simulink library "sm_car_testrig_utilities_lib"  (R2025a)
settings: Solver=VariableStepAuto  StartTime=0.0  StopTime=10.0  RelTol=1e-3
undefined symbols (not defined in the file): Maneuver, tire_radius, Vehicle, Visual, X, Y, Z
libraries: sm_lib x31, nesl_utility x18, fl_lib x3, $bdroot x3, Tire_Utilities x2, Surface_Profile_Axle2_KnC x2, simulink x2
(part 2 of 2)

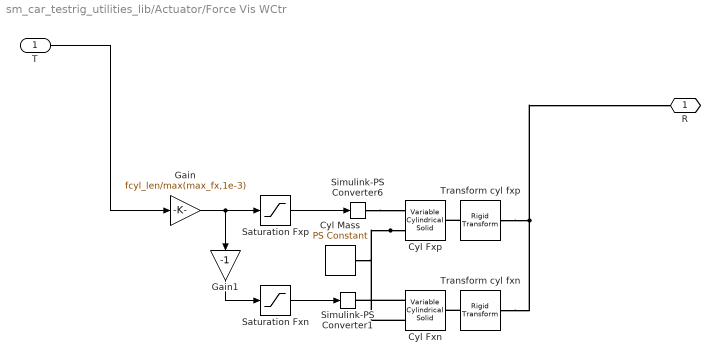
== system sm_car_testrig_utilities_lib/Actuator/Force Vis WCtr ==
  T : Inport
  Cyl Fxn : sm_lib/Body Elements/Variable Mass/Variable Cylindrical Solid  RadiusType=Constant  Radius=fcyl_rad  RadiusUnits=m  LengthType=ProvidedByInput  Length=1e-3  LengthUnits=m  MassType=ProvidedByInput  Density=1000  DensityUnits=kg/m^3  SenseRadius=off  SenseLength=off  SenseMass=off  SenseCenterOfMass=off  SenseInertiaMatrix=off  GraphicType=FromGeometry  MarkerShape=Sphere  MarkerSize=10  GraphicVisPropType=SimpleVisualProperties  GraphicDiffuseColor=fcyl_clr  GraphicOpacity=fcyl_opc  GraphicSpecularColor=[0.5 0.5 0.5 1.0]  GraphicAmbientColor=[0.15 0.15 0.15 1.0]  GraphicEmissiveColor=[0.0 0.0 0.0 1.0]  GraphicShininess=75
  Cyl Fxp : sm_lib/Body Elements/Variable Mass/Variable Cylindrical Solid  RadiusType=Constant  Radius=fcyl_rad  RadiusUnits=m  LengthType=ProvidedByInput  Length=1e-3  LengthUnits=m  MassType=ProvidedByInput  Density=1000  DensityUnits=kg/m^3  SenseRadius=off  SenseLength=off  SenseMass=off  SenseCenterOfMass=off  SenseInertiaMatrix=off  GraphicType=FromGeometry  MarkerShape=Sphere  MarkerSize=10  GraphicVisPropType=SimpleVisualProperties  GraphicDiffuseColor=fcyl_clr  GraphicOpacity=fcyl_opc  GraphicSpecularColor=[0.5 0.5 0.5 1.0]  GraphicAmbientColor=[0.15 0.15 0.15 1.0]  GraphicEmissiveColor=[0.0 0.0 0.0 1.0]  GraphicShininess=75
  Cyl Mass : fl_lib/Physical Signals/Sources/PS Constant  constant=1e-3
  Gain : Gain  Gain=fcyl_len/max(max_fx,1e-3)
  Gain1 : Gain  Gain=-1
  Saturation Fxn : Saturate  UpperLimit=inf  LowerLimit=0  ZeroCross=off
  Saturation Fxp : Saturate  UpperLimit=inf  LowerLimit=0  ZeroCross=off
  Simulink-PS Converter1 : nesl_utility/Simulink-PS Converter  PhysicalDomain=network_engine_domain  SubClassName=ps_input  LeftPortType=input  RightPortType=output  PseudoPeriodic=off  Frequencies=[]  NoiseDistribution=none  NoiseParameters=[]  Unit=1  AffineConversion=off  FilteringAndDerivatives=provide  SimscapeFilterOrder=1  InputFilterTimeConstant=0.001  UdotUserProvided=0
  Simulink-PS Converter6 : nesl_utility/Simulink-PS Converter  PhysicalDomain=network_engine_domain  SubClassName=ps_input  LeftPortType=input  RightPortType=output  PseudoPeriodic=off  Frequencies=[]  NoiseDistribution=none  NoiseParameters=[]  Unit=1  AffineConversion=off  FilteringAndDerivatives=provide  SimscapeFilterOrder=1  InputFilterTimeConstant=0.001  UdotUserProvided=0
  Transform cyl fxn : sm_lib/Frames and Transforms/Rigid Transform  RotationMethod=StandardAxis  FollAlignAxisA=+X  BaseAlignAxisA=+Y  FollAlignAxisB=+Y  BaseAlignAxisB=+Z  RotationStandardAxis=+Y  RotationAngle=-90  RotationAngleUnits=deg  RotationArbitraryAxis=[0 0 1]  RotationSequenceAxes=FollowerAxes  RotationSequence=XYX  RotationSequenceAngles=[0 0 0]  RotationSequenceAnglesUnits=deg  RotationMatrix=[1 0 0; 0 1 0; 0 0 1]  Quaternion=[1 0 0 0]  TranslationMethod=None  TranslationCartesianOffset=[0 0 0]  TranslationCartesianOffsetUnits=m  TranslationStandardAxis=+Z  TranslationStandardOffset=0  TranslationStandardOffsetUnits=m  TranslationROffset=0  TranslationROffsetUnits=m  TranslationThetaOffset=0  TranslationThetaOffsetUnits=deg  TranslationZOffset=0  TranslationZOffsetUnits=m
  Transform cyl fxp : sm_lib/Frames and Transforms/Rigid Transform  RotationMethod=StandardAxis  FollAlignAxisA=+X  BaseAlignAxisA=+Y  FollAlignAxisB=+Y  BaseAlignAxisB=+Z  RotationStandardAxis=+Y  RotationAngle=90  RotationAngleUnits=deg  RotationArbitraryAxis=[0 0 1]  RotationSequenceAxes=FollowerAxes  RotationSequence=XYX  RotationSequenceAngles=[0 0 0]  RotationSequenceAnglesUnits=deg  RotationMatrix=[1 0 0; 0 1 0; 0 0 1]  Quaternion=[1 0 0 0]  TranslationMethod=None  TranslationCartesianOffset=[0 0 0]  TranslationCartesianOffsetUnits=m  TranslationStandardAxis=+Z  TranslationStandardOffset=0  TranslationStandardOffsetUnits=m  TranslationROffset=0  TranslationROffsetUnits=m  TranslationThetaOffset=0  TranslationThetaOffsetUnits=deg  TranslationZOffset=0  TranslationZOffsetUnits=m
  R : PMIOPort  Side=Right
  wires:
  Saturation Fxn/1 -> Simulink-PS Converter1/1
  Saturation Fxp/1 -> Simulink-PS Converter6/1
  Gain/1 -> Saturation Fxp/1, Gain1/1
  T/1 -> Gain/1
  Gain1/1 -> Saturation Fxn/1
  connections:
  Cyl Fxp/LConn2 -- Cyl Fxn/LConn2 -- Cyl Mass/RConn1
  Transform cyl fxp/LConn1 -- Transform cyl fxn/LConn1 -- R/RConn1
  Simulink-PS Converter6/RConn1 -- Cyl Fxp/LConn1
  Transform cyl fxp/RConn1 -- Cyl Fxp/RConn1
  Cyl Fxn/LConn1 -- Simulink-PS Converter1/RConn1
  Transform cyl fxn/RConn1 -- Cyl Fxn/RConn1

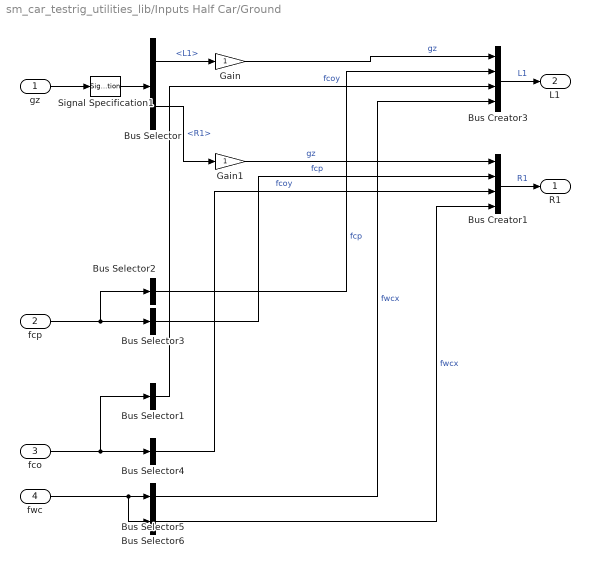
== system sm_car_testrig_utilities_lib/Inputs Half Car/Ground ==
  gz : Inport
  fcp : Inport  Port=2
  fco : Inport  Port=3
  fwc : Inport  Port=4
  Bus Creator1 : BusCreator  Inputs=4
  Bus Creator3 : BusCreator  Inputs=4
  Bus Selector : BusSelector  OutputSignals=L1,R1
  Bus Selector1 : BusSelector  OutputSignals=L1.fcoy  OutputAsBus=on
  Bus Selector2 : BusSelector  OutputSignals=L1.fx,L1.fy,L1.tz  OutputAsBus=on
  Bus Selector3 : BusSelector  OutputSignals=R1.fx,R1.fy,R1.tz  OutputAsBus=on
  Bus Selector4 : BusSelector  OutputSignals=R1.fcoy  OutputAsBus=on
  Bus Selector5 : BusSelector  OutputSignals=L1.fwcx  OutputAsBus=on
  Bus Selector6 : BusSelector  OutputSignals=R1.fwcx  OutputAsBus=on
  Gain : Gain
  Gain1 : Gain
  Signal Specification1 : SignalSpecification  Unit=m
  R1 : Outport  VectorParamsAs1DForOutWhenUnconnected=off
  L1 : Outport  Port=2  VectorParamsAs1DForOutWhenUnconnected=off
  wires:
  Bus Creator1/1 -> R1/1  "R1"
  Bus Creator3/1 -> L1/1  "L1"
  Signal Specification1/1 -> Bus Selector/1
  Bus Selector/1 -> Gain/1  "<L1>"
  gz/1 -> Signal Specification1/1
  Bus Selector/2 -> Gain1/1  "<R1>"
  Gain1/1 -> Bus Creator1/1  "gz"
  Gain/1 -> Bus Creator3/1  "gz"
  Bus Selector3/1 -> Bus Creator1/2  "fcp"
  fcp/1 -> Bus Selector2/1, Bus Selector3/1
  Bus Selector2/1 -> Bus Creator3/2  "fcp"
  fco/1 -> Bus Selector4/1, Bus Selector1/1
  Bus Selector1/1 -> Bus Creator3/3  "fcoy"
  Bus Selector4/1 -> Bus Creator1/3  "fcoy"
  fwc/1 -> Bus Selector6/1, Bus Selector5/1
  Bus Selector5/1 -> Bus Creator3/4  "fwcx"
  Bus Selector6/1 -> Bus Creator1/4  "fwcx"

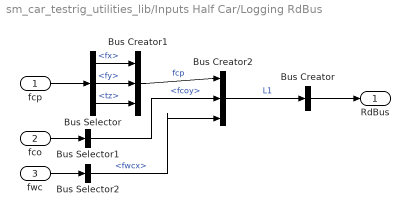
== system sm_car_testrig_utilities_lib/Inputs Half Car/Logging RdBus ==
  fcp : Inport
  fco : Inport  Port=2
  fwc : Inport  Port=3
  Bus Creator : BusCreator  Inputs=1
  Bus Creator1 : BusCreator  Inputs=3
  Bus Creator2 : BusCreator  Inputs=3
  Bus Selector : BusSelector  OutputSignals=L1.fx,L1.fy,L1.tz
  Bus Selector1 : BusSelector  OutputSignals=L1.fcoy
  Bus Selector2 : BusSelector  OutputSignals=L1.fwcx
  RdBus : Outport
  wires:
  Bus Selector/3 -> Bus Creator1/3  "<tz>"
  Bus Selector/2 -> Bus Creator1/2  "<fy>"
  Bus Selector/1 -> Bus Creator1/1  "<fx>"
  Bus Creator2/1 -> Bus Creator/1  "L1"
  Bus Creator1/1 -> Bus Creator2/1  "fcp"
  Bus Creator/1 -> RdBus/1
  fcp/1 -> Bus Selector/1
  fco/1 -> Bus Selector1/1
  Bus Selector1/1 -> Bus Creator2/2  "<fcoy>"
  fwc/1 -> Bus Selector2/1
  Bus Selector2/1 -> Bus Creator2/3  "<fwcx>"

== system sm_car_testrig_utilities_lib/Inputs Half Car/Steering ==
  Off : Subsystem  VariantControl=Off
  On : Subsystem  VariantControl=On
  qStr : Outport
  xRk : Outport  Port=2

== system sm_car_testrig_utilities_lib/Inputs Quarter Car/Logging RdBus ==
  L1 : Inport
  Bus Creator : BusCreator  Inputs=1
  Bus Creator1 : BusCreator  Inputs=3
  Bus Creator2 : BusCreator  Inputs=1
  Bus Selector : BusSelector  OutputSignals=L1.fx,L1.fy,L1.tz
  RdBus : Outport
  wires:
  L1/1 -> Bus Selector/1
  Bus Creator/1 -> RdBus/1
  Bus Creator1/1 -> Bus Creator2/1  "fcp"
  Bus Creator2/1 -> Bus Creator/1  "L1"
  Bus Selector/1 -> Bus Creator1/1  "<fx>"
  Bus Selector/2 -> Bus Creator1/2  "<fy>"
  Bus Selector/3 -> Bus Creator1/3  "<tz>"

== system sm_car_testrig_utilities_lib/Inputs Quarter Car/Steering ==
  Off : Subsystem  VariantControl=Off
  On : Subsystem  VariantControl=On
  qStr : Outport
  xRk : Outport  Port=2

== system sm_car_testrig_utilities_lib/Inputs Half Car/Steering/Off ==
  Constant : Constant  Value=0
  qStr : Outport
  xRk : Outport  Port=2
  wires:
  Constant/1 -> qStr/1, xRk/1

== system sm_car_testrig_utilities_lib/Inputs Half Car/Steering/On ==
  note: More logic would be needed to run KnC tests on rack-driven steering systems. For now we set it to 0 as it is not used to drive the half-car testrig.
  Gain : Gain  Gain=0
  Steer to Rack : Lookup_n-D  Commented=on  NumberOfTableDimensions=1  BreakpointsForDimension1=Vehicle.Chassis.SuspA1.Steer.Ratio_Table.aWheel.Value  Table=Vehicle.Chassis.SuspA1.Steer.Ratio_Table.xRack.Value  InternalRulePriority=Speed  RndMeth=Simplest
  qSteer : simulink/Sources/Repeating Sequence  rep_seq_t=Maneuver.Steer.t.Value  rep_seq_y=Maneuver.Steer.aWheel.Value
  qStr : Outport
  xRk : Outport  Port=2
  wires:
  Gain/1 -> xRk/1
  qSteer/1 -> Gain/1, qStr/1

== system sm_car_testrig_utilities_lib/Inputs Quarter Car/Steering/Off ==
  Constant : Constant  Value=0
  qStr : Outport
  xRk : Outport  Port=2
  wires:
  Constant/1 -> xRk/1, qStr/1

== system sm_car_testrig_utilities_lib/Inputs Quarter Car/Steering/On ==
  Steer to Rack : Lookup_n-D  NumberOfTableDimensions=1  BreakpointsForDimension1=Vehicle.Chassis.SuspA1.Steer.Ratio_Table.aWheel.Value  Table=Vehicle.Chassis.SuspA1.Steer.Ratio_Table.xRack.Value  InternalRulePriority=Speed  RndMeth=Simplest
  qSteer : simulink/Sources/Repeating Sequence  rep_seq_t=Maneuver.Steer.t.Value  rep_seq_y=Maneuver.Steer.aWheel.Value
  qStr : Outport
  xRk : Outport  Port=2
  wires:
  qSteer/1 -> qStr/1, Steer to Rack/1
  Steer to Rack/1 -> xRk/1
